simulink model "PruebasKUF"  (R2026a)
settings: Solver=VariableStepAuto  StopTime=50  MaxStep=0.01
values from neighbouring files (symbols this model uses):
  B = -c.b*I/r^2    [ComparacionKUF.m]
  g = 9.81    [ComparacionKUF.m]    (also in DespejeKuf.m)
  I = 3.2*382.232e-7    (= 0.00012231424)    [ComparacionKUF.m]
  kuf = fit_linear(1)    [ComparacionKUF.m]
  kuf_0 = fit_linear(2)    [ComparacionKUF.m]
  kuf_a = 0.0642    [ComparacionKUF.m]
  kuf_b = 0.0046    [ComparacionKUF.m]
  kuf_c = -0.0647    [ComparacionKUF.m]
  kuf_d = -0.0187    [ComparacionKUF.m]
  lc = 40.67e-3    (= 0.04067)    [ComparacionKUF.m]    (also in DespejeKuf.m = 0.040677)
  m = 30.00e-3    (= 0.03)    [ComparacionKUF.m]    (also in DespejeKuf.m)
  r = 135.0e-3    (= 0.135)    [ComparacionKUF.m]    (also in DespejeKuf.m)
libraries: simulink x2
settings Model: Creator=sslan  LastModifiedBy=leonardoa29

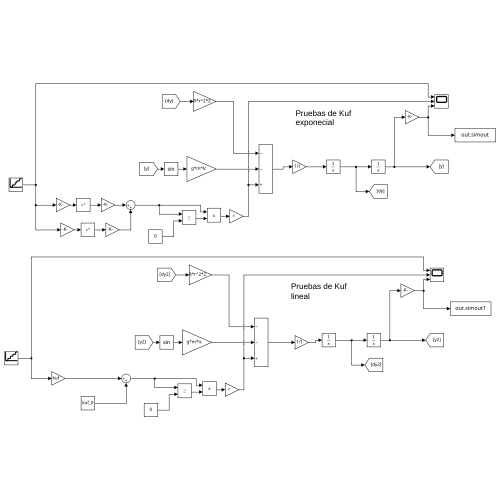
[thumbnail: Simulink's stored preview of the top-level diagram]
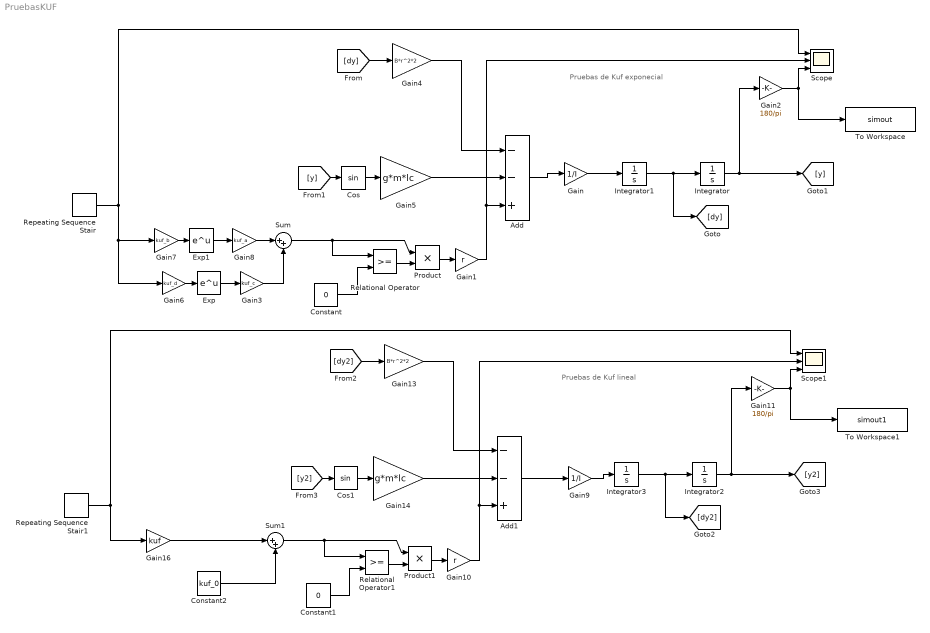
== system PruebasKUF ==
  note: Pruebas de Kuf exponecial
  note: Pruebas de Kuf lineal
  Add : Sum  Inputs=--+
  Add1 : Sum  Inputs=--+
  Constant : Constant  Value=0
  Constant1 : Constant  Value=0
  Constant2 : Constant  Value=kuf_0
  Cos : Trigonometry
  Cos1 : Trigonometry
  Exp : Math
  Exp1 : Math
  Gain : Gain  Gain=1/I
  Gain1 : Gain  Gain=r
  Gain10 : Gain  Gain=r
  Gain11 : Gain  Gain=180/pi
  Gain13 : Gain  Gain=B*r^2*2
  Gain14 : Gain  Gain=g*m*lc
  Gain16 : Gain  Gain=kuf
  Gain2 : Gain  Gain=180/pi
  Gain3 : Gain  Gain=kuf_c
  Gain4 : Gain  Gain=B*r^2*2
  Gain5 : Gain  Gain=g*m*lc
  Gain6 : Gain  Gain=kuf_d
  Gain7 : Gain  Gain=kuf_b
  Gain8 : Gain  Gain=kuf_a
  Gain9 : Gain  Gain=1/I
  Integrator{,1..3} (4 alike) : Integrator
  Product : Product
  Product1 : Product
  Relational Operator : RelationalOperator  OutDataTypeStr=boolean  RndMeth=Simplest  InputSameDT=off
  Relational Operator1 : RelationalOperator  OutDataTypeStr=boolean  RndMeth=Simplest  InputSameDT=off
  Repeating Sequence Stair : simulink/Sources/Repeating Sequence Stair  OutValues=repeating_sequence  tsamp=step_interval  OutMin=[]  OutMax=[]  OutDataTypeStr=double  OutputDataTypeScalingMode=double  OutDataType=fixdt(0,8)  ConRadixGroup=Best Precision: Vector-wise  OutScaling=2^-12
  Repeating Sequence Stair1 : simulink/Sources/Repeating Sequence Stair  OutValues=repeating_sequence  tsamp=step_interval  OutMin=[]  OutMax=[]  OutDataTypeStr=double  OutputDataTypeScalingMode=double  OutDataType=fixdt(0,8)  ConRadixGroup=Best Precision: Vector-wise  OutScaling=2^-12
  Scope : Scope  NumInputPorts=3
      settings: ActiveDisplayYMinimum=-1.0572635942699053  ActiveDisplayYMaximum=9.51537234842915
  Scope1 : Scope  NumInputPorts=3
      settings: ActiveDisplayYMinimum=-1.2385894560506807  ActiveDisplayYMaximum=11.147305104456128
  Sum : Sum  Inputs=|++
  Sum1 : Sum  Inputs=|++
  To Workspace : ToWorkspace  VariableName=simout  SaveFormat=Timeseries  SampleTime=-1
  To Workspace1 : ToWorkspace  VariableName=simout1  SaveFormat=Timeseries  SampleTime=-1
  wires:
  Gain5/1 -> Add/2
  Cos/1 -> Gain5/1
  Integrator/1 -> [y], Gain2/1
  Gain/1 -> Integrator1/1
  [y] -> Cos/1
  Integrator1/1 -> [dy], Integrator/1
  [dy] -> Gain4/1
  Gain2/1 -> Scope/3, To Workspace/1
  Repeating Sequence Stair/1 -> Gain6/1, Gain7/1, Scope/1
  Gain6/1 -> Exp/1
  Exp/1 -> Gain3/1
  Exp1/1 -> Gain8/1
  Gain7/1 -> Exp1/1
  Gain8/1 -> Sum/1
  Gain3/1 -> Sum/2
  Constant/1 -> Relational Operator/2
  Sum/1 -> Product/1, Relational Operator/1
  Gain1/1 -> Add/3, Scope/2
  Relational Operator/1 -> Product/2
  Gain4/1 -> Add/1
  Product/1 -> Gain1/1
  Add/1 -> Gain/1
  [dy2] -> Gain13/1
  Gain16/1 -> Sum1/1
  Gain11/1 -> Scope1/3, To Workspace1/1
  Constant1/1 -> Relational Operator1/2
  Integrator2/1 -> [y2], Gain11/1
  Gain14/1 -> Add1/2
  Add1/1 -> Gain9/1
  Gain13/1 -> Add1/1
  [y2] -> Cos1/1
  Integrator3/1 -> [dy2], Integrator2/1
  Sum1/1 -> Product1/1, Relational Operator1/1
  Relational Operator1/1 -> Product1/2
  Gain9/1 -> Integrator3/1
  Cos1/1 -> Gain14/1
  Gain10/1 -> Add1/3, Scope1/2
  Repeating Sequence Stair1/1 -> Gain16/1, Scope1/1
  Product1/1 -> Gain10/1
  Constant2/1 -> Sum1/2
